simulink model "speed_measurement"  (R2026a)
settings: Solver=FixedStepAuto  StopTime=inf  EnableMultiTasking=on
libraries: arduinosensorlib x1, arduinolib x1
settings Model: SILPILModeSetting=veronly  ExtModeTrigDuration=2  Creator=cas_g  LastModifiedBy=00782620
settings HardwareCC: ProdBitPerInt=16.0  ProdBitPerPointer=16.0  ProdBitPerSizeT=16.0  ProdBitPerPtrDiffT=16.0  ProdWordSize=8.0  ProdHWDeviceType=Atmel->AVR
settings RTWCC: SystemTargetFile=ert.tlc  HardwareBoard=Arduino Uno  TLCOptions=-aInlineSetEventsForThisBaseRateFcn=TLC_FALSE -aSuppressMultiTaskScheduler=TLC_FALSE -aRateBasedStepFcn=1  Toolchain=Arduino AVR  BuildConfiguration=Faster Runs  Description=Embedded Coder
settings ERTTargetCC: ExtModeTransport=3.0  ExtModeAutomaticAllocSize=off  ExtModeStaticAllocSize=250.0  SupportContinuousTime=on  SupportVariableSizeSignals=on

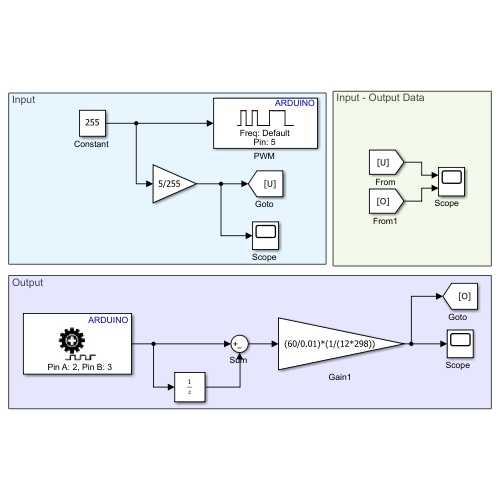
[thumbnail: Simulink's stored preview of the top-level diagram]
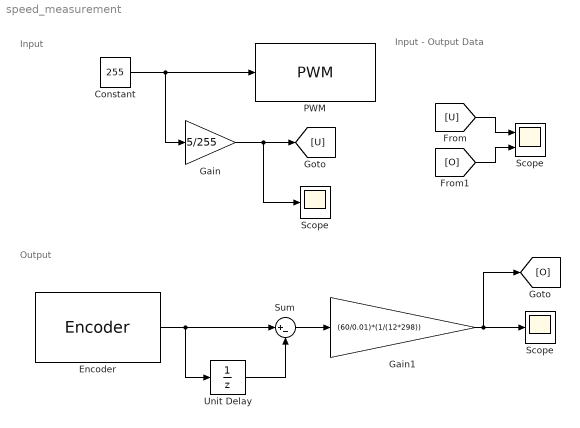
== system speed_measurement ==
  note: Input - Output Data
  note: Input
  note: Output
  "Constant " : Constant  Value=255
  Encoder : arduinosensorlib/Encoder  InputA=2  InputB=3  Mode=No reset  SampleTime=0.01
  Gain : Gain  Gain=5/255
  "Gain1 " : Gain  Gain=(60/0.01)*(1/(12*298))
  "PWM " : arduinolib/PWM  pinNumber=5  frequencyType=Default  desiredFrequency=490.2  achievableFrequency=490.2
  "Scope " : Scope
  "Scope  " : Scope
      settings: ActiveDisplayYMinimum=-110.94798660115339  ActiveDisplayYMaximum=-108.85067116445862
  "Scope    " : Scope  NumInputPorts=2
      settings: ActiveDisplayYMinimum=-8.2172818821854854  ActiveDisplayYMaximum=123.9555369396694  DataLoggingVariableName=ScopeData2
  "Sum " : Sum  Inputs=|+-
  Unit Delay : UnitDelay  SampleTime=-1
  wires:
  "Constant "/1 -> Gain/1, "PWM "/1
  Gain/1 -> "Scope "/1, [U]
  Encoder/1 -> "Sum "/1, Unit Delay/1
  "Gain1 "/1 -> [O], "Scope  "/1
  [U] -> "Scope    "/1
  [O] -> "Scope    "/2
  "Sum "/1 -> "Gain1 "/1
  Unit Delay/1 -> "Sum "/2
